simulink model "ball_balancing_omni3_multibody_lqi_rev2_r2024b"  (R2024b)
settings: Solver=VariableStepAuto  StartTime=0.0  StopTime=5  MaxStep=1e-3  MinStep=1e-6  RelTol=ballbotParams.simulation.relativeTolerance
PreLoadFcn:
  | if ~exist('ballbotParams','var'), ballbotParams = ballbotRev1Parameters; end
InitFcn:
  | if ~exist('ballbotParams','var') || ~isfield(ballbotParams,'parameterSource') || ballbotParams.parameterSource ~= "ballbotRev1Parameters" || ~isfield(ballbotParams,'controller') || ~isfield(ballbotParams,'estimator') || ~isfield(ballbotParams.controller,'torqueDrive') || ~isfield(ballbotParams.controller.torqueDrive,'propulsionGain') || ~isfield(ballbotParams.estimator,'truthDelaySteps') || ~isfield(ballbotParams.controller.torqueLqi,'robustness'), ballbotParams = ballbotRev1Parameters; end
  | % ballbotRev1RuntimeApply: re-apply runtime solver/driver/plant settings on every sim start.
  | clear functions;
  | ballbotRev1SimConfig;
  | if exist('ballbotParams','var'), ballbotRev1PlantAugment(bdroot, ballbotParams); end
values from neighbouring files (symbols this model uses):
  N = 0    [ballbotRollingResistance.m]
  s = result.spec    [ballbotBenchmark.m]
undefined symbols (not defined in the file or in its folder): ballbotCustomFriction, ballbotEstimatorUpdate, ballbotEulerToQuaternion, ballbotImuFromJoint, ballbotLqiControllerUpdateRev2, ballbotLqiFeedbackState, ballbotMdd3aGateDrive, ballbotParams, ballbotPoseFromJoint, ballbotRev1CommandProfile, ballbotRollingResistance, ballbotRoverInitialPosition, ballbotShaftFrictionTorque, ballbotTruthGate, ballbotWheelRateFromDisplacement, ballbotWheelServoDutyStep, X, Y, Z
libraries: nesl_utility x54, sm_lib x28, fl_lib x21, ee_lib x6
(part 3 of 3)

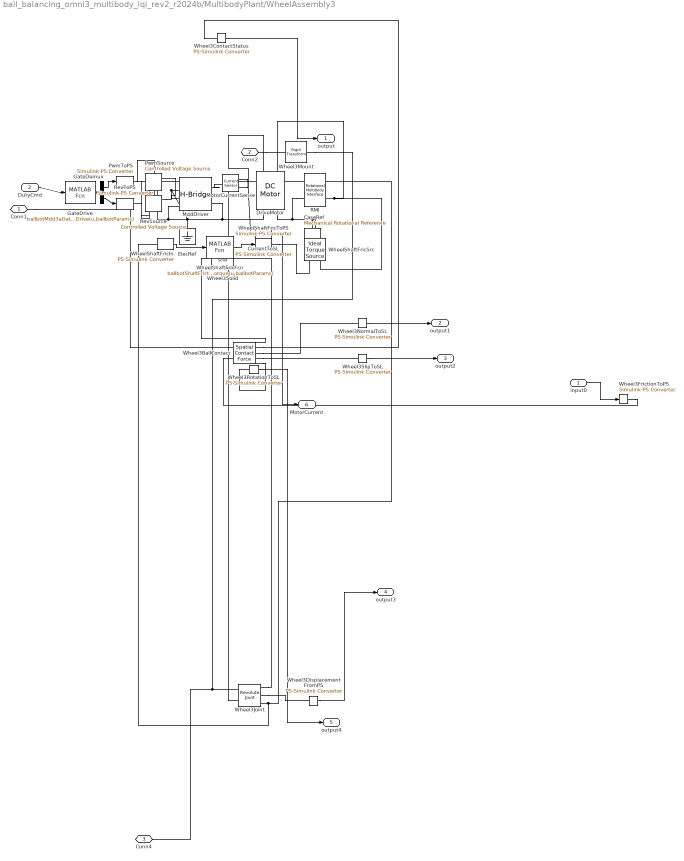
== system ball_balancing_omni3_multibody_lqi_rev2_r2024b/MultibodyPlant/WheelAssembly3 ==
  input0 : Inport
  DutyCmd : Inport  Port=2
  CaseRef : fl_lib/Mechanical/Rotational Elements/Mechanical Rotational Reference
  CurrentToSL : nesl_utility/PS-Simulink Converter  PhysicalDomain=network_engine_domain  SubClassName=ps_output  LeftPortType=input  RightPortType=output  PseudoPeriodic=off  Frequencies=[]  VectorFormat=inherit  Unit=A  AffineConversion=off
  DriveMotor : ee_lib/Electromechanical/Brushed Motors/DC Motor  field_option=ee.enum.field_option.pm  Rf=100 Ohm  Lf=1 H  Laf=0.15 H  If0=0 A  parameterization=ee.enum.dcparam_option.circuit_param  Ra=ballbotParams.motor.armatureResistance Ohm  La=ballbotParams.motor.armatureInductance H  emf_or_torque=ee.enum.emf_or_torque.ki  Kv=0.072e-3 V/rpm  Ki=ballbotParams.motor.torqueConstant N*m/A  T_stall=0.24e-3 N*m  w_max=19100 rpm  w_rated=15000 rpm  P_rated=0.08 W  V_rated=1.5 V  lam_param=ee.enum.lam_param.damping  i_noload=0 A  V_i_noload=1.5 V  J=ballbotParams.motor.equivalentInertia kg*m^2  lam=ballbotParams.motor.viscousFriction*ballbotParams.motor.viscousShare N*m*s/rad  speed0=0 rpm  alpha=3.93e-3 1/K  Tmeas=25 degC  thermal_mass=100 J/K  initial_temperature=25 degC
  ElecRef : fl_lib/Electrical/Electrical Elements/Electrical Reference
  GateDemux : Demux  Outputs=2
  GateDrive : MATLABFcn  MATLABFcn=ballbotMdd3aGateDrive(u,ballbotParams)  OutputDimensions=2
  MddDriver : ee_lib/Semiconductors & Converters/Converters/H-Bridge  pwm_or_av=ee.enum.pwm_or_av.averaged  discontinuous=ee.enum.current_profile.continuous  freewheeling_mode=ee.enum.converters.freewheeling_mode.one_switch_one_diode  Rload=10 Ohm  Lload=1e-5 H  F=ballbotParams.driver.pwmFrequency Hz  supply_ports=ee.enum.supply_ports.hidesupply  regenerative_braking_mode=ee.enum.converters.regenerative_braking_mode.always_enabled  Venable=ballbotParams.driver.enableThresholdVoltage V  Vmax=ballbotParams.driver.logicHighVoltage V  Vreverse=ballbotParams.driver.reverseThresholdVoltage V  Vbrake=ballbotParams.driver.brakeThresholdVoltage V  Vm=ballbotParams.driver.supplyVoltage V  Ron=ballbotParams.driver.bridgeOnResistance Ohm  Don=0.05 Ohm  Goff=1e-6 S  Tmeas=298.15 K  Ron2=0.1 Ohm  Don2=0.05 Ohm  Tmeas2=398.15 K  thermal_mass=100 J/K  initial_temperature=298.15 K
  MotorCurrentSense : fl_lib/Electrical/Electrical Sensors/Current Sensor
  PwmSource : fl_lib/Electrical/Electrical Sources/Controlled Voltage Source
  PwmToPS : nesl_utility/Simulink-PS Converter  PhysicalDomain=network_engine_domain  SubClassName=ps_input  LeftPortType=input  RightPortType=output  PseudoPeriodic=off  Frequencies=[]  NoiseDistribution=none  NoiseParameters=[]  Unit=1  AffineConversion=off  FilteringAndDerivatives=provide  SimscapeFilterOrder=1  InputFilterTimeConstant=0.001  UdotUserProvided=0
  RMI : fl_lib/Mechanical/Multibody Interfaces/Rotational Multibody Interface
  RevSource : fl_lib/Electrical/Electrical Sources/Controlled Voltage Source
  RevToPS : nesl_utility/Simulink-PS Converter  PhysicalDomain=network_engine_domain  SubClassName=ps_input  LeftPortType=input  RightPortType=output  PseudoPeriodic=off  Frequencies=[]  NoiseDistribution=none  NoiseParameters=[]  Unit=1  AffineConversion=off  FilteringAndDerivatives=provide  SimscapeFilterOrder=1  InputFilterTimeConstant=0.001  UdotUserProvided=0
  Wheel3BallContact : sm_lib/Forces and Torques/Spatial Contact Force  SenseSeparationDistance=off  NormalForceType=SmoothSpringDamper  NormalStiffness=ballbotParams.contact.wheelBall.normalStiffness  NormalStiffnessUnits=N/m  NormalDamping=ballbotParams.contact.wheelBall.normalDamping  NormalDampingUnits=N/(m/s)  NormalTransitionRegionWidth=ballbotParams.contact.wheelBall.relaxedTransitionWidth  NormalTransitionRegionWidthUnits=m  FrictionType=ProvidedByInput  CoefficientOfStaticFriction=ballbotParams.contact.wheelBall.staticFriction  CoefficientOfDynamicFriction=ballbotParams.contact.wheelBall.dynamicFriction  FrictionalCriticalVelocity=ballbotParams.contact.wheelBall.criticalVelocity  FrictionalCriticalVelocityUnits=m/s  SenseContactSignal=on  SensePenetrationDepth=off  SenseNormalVelocity=off  SenseTangentialVelocity=on  SensingForceTorqueDirection=BaseOnFollower  SensingForceTorqueResolutionFrame=ContactFrame  SenseNormalForce=off  SenseNormalForceMagnitude=on  SenseNormalTorque=off  SenseFrictionalForce=off  SenseFrictionalForceMagnitude=off  SenseFrictionalTorque=off  SenseTotalForce=off  SenseTotalTorque=off  SenseContactBaseRotation=off  SenseContactBaseTranslation=off  SenseContactFollowerRotation=on  SenseContactFollowerTranslation=off  ZeroCrossDetectContactStartAndEnd=on
  Wheel3ContactStatus : nesl_utility/PS-Simulink Converter  PhysicalDomain=network_engine_domain  SubClassName=ps_output  LeftPortType=input  RightPortType=output  PseudoPeriodic=off  Frequencies=[]  VectorFormat=inherit  Unit=1  AffineConversion=off
  Wheel3DisplacementFromPS : nesl_utility/PS-Simulink Converter  PhysicalDomain=network_engine_domain  SubClassName=ps_output  LeftPortType=input  RightPortType=output  PseudoPeriodic=off  Frequencies=[]  VectorFormat=inherit  Unit=rad  AffineConversion=off
  Wheel3FrictionToPS : nesl_utility/Simulink-PS Converter  PhysicalDomain=network_engine_domain  SubClassName=ps_input  LeftPortType=input  RightPortType=output  PseudoPeriodic=off  Frequencies=[]  NoiseDistribution=none  NoiseParameters=[]  Unit=N  AffineConversion=off  FilteringAndDerivatives=provide  SimscapeFilterOrder=1  InputFilterTimeConstant=0.001  UdotUserProvided=0
  Wheel3Joint : sm_lib/Joints/Revolute Joint  JointMode=Normal  CompositeWrenchDir=FollowerOnBase  CompositeWrenchFrame=BaseFrame  SenseConstraintForce=off  SenseConstraintTorque=off  SenseTotalForce=off  SenseTotalTorque=off  PositionTargetSpecify=off  PositionTargetPriority=High  PositionTargetValue=0  PositionTargetValueUnits=deg  VelocityTargetSpecify=off  VelocityTargetPriority=High  VelocityTargetValue=0  VelocityTargetValueUnits=deg/s  EquilibriumPosition=0  EquilibriumPositionUnits=deg  SpringStiffness=0  SpringStiffnessUnits=N*m/deg  DampingCoefficient=0  DampingCoefficientUnits=N*m/(deg/s)  LowerLimitSpecify=off  LowerLimitBound=-90  LowerLimitBoundUnits=deg  LowerLimitStiffness=1e4  LowerLimitStiffnessUnits=N*m/deg  LowerLimitDamping=10  LowerLimitDampingUnits=N*m/(deg/s)  LowerLimitTransitionRegionWidth=0.1  LowerLimitTransitionRegionWidthUnits=deg  UpperLimitSpecify=off  UpperLimitBound=90  UpperLimitBoundUnits=deg  UpperLimitStiffness=1e4  UpperLimitStiffnessUnits=N*m/deg  UpperLimitDamping=10  UpperLimitDampingUnits=N*m/(deg/s)  UpperLimitTransitionRegionWidth=0.1  UpperLimitTransitionRegionWidthUnits=deg  TorqueActuationMode=InputTorque  MotionActuationMode=ComputedMotion  SensePosition=on  SenseVelocity=on  SenseAcceleration=off  SenseTorqueForce=off  SenseLowerLimitTorqueForce=off  SenseUpperLimitTorqueForce=off
  Wheel3Mount : sm_lib/Frames and Transforms/Rigid Transform  RotationMethod=RotationMatrix  FollAlignAxisA=+X  BaseAlignAxisA=+Y  FollAlignAxisB=+Y  BaseAlignAxisB=+Z  RotationStandardAxis=+Z  RotationAngle=0  RotationAngleUnits=deg  RotationArbitraryAxis=[0 0 1]  RotationSequenceAxes=FollowerAxes  RotationSequence=XYX  RotationSequenceAngles=[0 0 0]  RotationSequenceAnglesUnits=deg  RotationMatrix=[ballbotParams.wheel.geometry.rollingBody(:,3),-ballbotParams.wheel.geometry.normalBody(:,3),ballbotParams.wheel.geometry.axleBody(:,3)]  Quaternion=[1 0 0 0]  TranslationMethod=Cartesian  TranslationCartesianOffset=ballbotParams.wheel.geometry.centerFromBody(:,3)'  TranslationCartesianOffsetUnits=m  TranslationStandardAxis=+Z  TranslationStandardOffset=0  TranslationStandardOffsetUnits=m  TranslationROffset=0  TranslationROffsetUnits=m  TranslationThetaOffset=0  TranslationThetaOffsetUnits=deg  TranslationZOffset=0  TranslationZOffsetUnits=m
  Wheel3NormalToSL : nesl_utility/PS-Simulink Converter  PhysicalDomain=network_engine_domain  SubClassName=ps_output  LeftPortType=input  RightPortType=output  PseudoPeriodic=off  Frequencies=[]  VectorFormat=inherit  Unit=N  AffineConversion=off
  Wheel3RotationToSL : nesl_utility/PS-Simulink Converter  PhysicalDomain=network_engine_domain  SubClassName=ps_output  LeftPortType=input  RightPortType=output  PseudoPeriodic=off  Frequencies=[]  VectorFormat=inherit  Unit=1  AffineConversion=off
  Wheel3SlipToSL : nesl_utility/PS-Simulink Converter  PhysicalDomain=network_engine_domain  SubClassName=ps_output  LeftPortType=input  RightPortType=output  PseudoPeriodic=off  Frequencies=[]  VectorFormat=inherit  Unit=m/s  AffineConversion=off
  Wheel3Solid : sm_lib/Body Elements/Cylindrical Solid  CylinderRadius=ballbotParams.wheel.radius  CylinderRadiusUnits=m  CylinderLength=ballbotParams.wheel.width  CylinderLengthUnits=m  ExportEntireGeometry=on  InertiaType=CalculateFromGeometry  BasedOnType=Mass  Density=1000  DensityUnits=kg/m^3  Mass=ballbotParams.wheel.mass  MassUnits=kg  CenterOfMass=[0 0 0]  CenterOfMassUnits=m  MomentsOfInertia=[1 1 1]  MomentsOfInertiaUnits=kg*m^2  ProductsOfInertia=[0 0 0]  ProductsOfInertiaUnits=kg*m^2  GraphicType=FromGeometry  MarkerShape=Sphere  MarkerSize=10  GraphicVisPropType=SimpleVisualProperties  GraphicDiffuseColor=[0.5 0.5 0.5]  GraphicOpacity=1  GraphicSpecularColor=[0.5 0.5 0.5 1.0]  GraphicAmbientColor=[0.15 0.15 0.15 1.0]  GraphicEmissiveColor=[0.0 0.0 0.0 1.0]  GraphicShininess=75  DoExposeReferenceFrame=on  SerializedFrames=<Frames/>
  WheelShaftFricFcn : MATLABFcn  MATLABFcn=ballbotShaftFrictionTorque(u,ballbotParams)
  WheelShaftFricIn : nesl_utility/PS-Simulink Converter  PhysicalDomain=network_engine_domain  SubClassName=ps_output  LeftPortType=input  RightPortType=output  PseudoPeriodic=off  Frequencies=[]  VectorFormat=inherit  Unit=rad/s  AffineConversion=off
  WheelShaftFricSrc : fl_lib/Mechanical/Mechanical Sources/Ideal Torque Source
  WheelShaftFricToPS : nesl_utility/Simulink-PS Converter  PhysicalDomain=network_engine_domain  SubClassName=ps_input  LeftPortType=input  RightPortType=output  PseudoPeriodic=off  Frequencies=[]  NoiseDistribution=none  NoiseParameters=[]  Unit=N*m  AffineConversion=off  FilteringAndDerivatives=provide  SimscapeFilterOrder=1  InputFilterTimeConstant=0.001  UdotUserProvided=0
  Conn1 : PMIOPort  Side=Left
  Conn2 : PMIOPort  Port=2  Side=Left
  Conn4 : PMIOPort  Port=3  Side=Left
  output : Outport
  output1 : Outport  Port=2
  output2 : Outport  Port=3
  output3 : Outport  Port=4
  output4 : Outport  Port=5
  MotorCurrent : Outport  Port=6
  wires:
  Wheel3DisplacementFromPS/1 -> output3/1
  input0/1 -> Wheel3FrictionToPS/1
  Wheel3RotationToSL/1 -> output4/1
  Wheel3ContactStatus/1 -> output/1
  Wheel3SlipToSL/1 -> output2/1
  Wheel3NormalToSL/1 -> output1/1
  DutyCmd/1 -> GateDrive/1
  GateDrive/1 -> GateDemux/1
  GateDemux/1 -> PwmToPS/1
  GateDemux/2 -> RevToPS/1
  CurrentToSL/1 -> MotorCurrent/1
  WheelShaftFricIn/1 -> WheelShaftFricFcn/1
  WheelShaftFricFcn/1 -> WheelShaftFricToPS/1
  connections:
  Wheel3FrictionToPS/RConn1 -- Wheel3BallContact/LConn2
  Wheel3BallContact/RConn2 -- Wheel3ContactStatus/LConn1
  Wheel3Joint/RConn1 -- Wheel3Solid/RConn1
  Wheel3BallContact/RConn4 -- Wheel3SlipToSL/LConn1
  Wheel3Solid/LConn1 -- Wheel3BallContact/RConn1
  Wheel3BallContact/RConn5 -- Wheel3RotationToSL/LConn1
  Wheel3BallContact/RConn3 -- Wheel3NormalToSL/LConn1
  Wheel3Joint/RConn2 -- Wheel3DisplacementFromPS/LConn1
  Conn1/RConn1 -- Wheel3BallContact/LConn1
  PwmToPS/RConn1 -- PwmSource/RConn1
  RevToPS/RConn1 -- RevSource/RConn1
  PwmSource/LConn1 -- MddDriver/LConn1
  RevSource/LConn1 -- MddDriver/LConn3
  RevSource/RConn2 -- DriveMotor/RConn1 -- MddDriver/RConn2 -- ElecRef/LConn1 -- PwmSource/RConn2 -- MddDriver/LConn2 -- MddDriver/LConn4
  MddDriver/RConn1 -- MotorCurrentSense/LConn1
  MotorCurrentSense/RConn2 -- DriveMotor/LConn1
  MotorCurrentSense/RConn1 -- CurrentToSL/LConn1
  RMI/RConn2 -- DriveMotor/LConn2 -- WheelShaftFricSrc/RConn2
  RMI/LConn2 -- CaseRef/LConn1 -- WheelShaftFricSrc/LConn1 -- DriveMotor/RConn2
  RMI/RConn1 -- Wheel3Joint/RConn3 -- WheelShaftFricIn/LConn1
  RMI/LConn1 -- Wheel3Joint/LConn2
  Wheel3Mount/RConn1 -- Wheel3Joint/LConn1 -- Conn4/RConn1
  Conn2/RConn1 -- Wheel3Mount/LConn1
  WheelShaftFricToPS/RConn1 -- WheelShaftFricSrc/RConn1
